simulink model "SvpwmComparisonTest"  (R2026b)
settings: Solver=FixedStepDiscrete  StopTime=svpwmTest.StopTime  FixedStep=svpwmTest.Ts
PostLoadFcn:
  | svpwmDir=fileparts(get_param(bdroot,'FileName'));addpath(fullfile(svpwmDir,'seven_segment'),fullfile(svpwmDir,'five_segment'),fullfile(svpwmDir,'..','..','parameter'));assignin(get_param(bdroot,'ModelWorkspace'),'svpwmTest',svpwm_test_parameters());clear svpwmDir;
model workspace (MAT data in the model file):
  svpwmTest.Ts = 0.0001
  svpwmTest.Stimulus = [0  16.6276877527  9.6  48; 0.0001  1.17566092718e-15  19.2  48; 0.0002  -16.6276877527  9.6  48; 0.0003  -16.6276877527  -9.6  48; 0.0004  -3.52698278154e-15  -19.2  48; 0.0005  16.6276877527  -9.6  48; 0.0006  8.31384387633  4.8  24; 0.0007  5.87830463591e-16  9.6  24; 0.0008  -8.31384387633  4.8  24; 0.0009  -8.31384387633  -4.8  24; 0.001  -1.76349139077e-15  -9.6  24; 0.0011  8.31384387633  -4.8  24; 0.0012  0  0  48; 0.0013  48  0  48]
  svpwmTest.StopTime = 0.0013
libraries: SvpwmFiveSegment x1, SvpwmSevenSegment x1
settings Model: Creator=24322  LastModifiedBy=24322

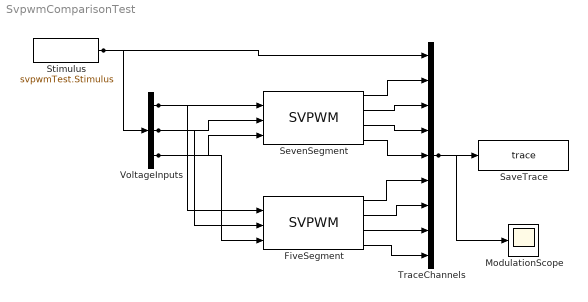
== system SvpwmComparisonTest ==
  FiveSegment : SvpwmFiveSegment/SVPWM  SystemSampleTime=-1  VariantActivationTime=update diagram  EmptyChoice=off  PassThrough=off  PassThroughVariantControl=(default)  EmptyChoiceVariantControl=(default)  AllowFlexibleInterface=on  Latency=0  AutoFrameSizeCalculation=off
  ModulationScope : Scope
  SaveTrace : ToWorkspace  VariableName=trace  SaveFormat=Structure With Time  SampleTime=-1
  SevenSegment : SvpwmSevenSegment/SVPWM  SystemSampleTime=-1  VariantActivationTime=update diagram  EmptyChoice=off  PassThrough=off  PassThroughVariantControl=(default)  EmptyChoiceVariantControl=(default)  AllowFlexibleInterface=on  Latency=0  AutoFrameSizeCalculation=off
  Stimulus : FromWorkspace  VariableName=svpwmTest.Stimulus  SampleTime=svpwmTest.Ts  Interpolate=off  OutputAfterFinalValue=Holding final value
  TraceChannels : Mux  Inputs=9
  VoltageInputs : Demux  Outputs=3
  wires:
  FiveSegment/4 -> TraceChannels/9
  SevenSegment/4 -> TraceChannels/5
  FiveSegment/3 -> TraceChannels/8
  SevenSegment/3 -> TraceChannels/4
  FiveSegment/2 -> TraceChannels/7
  SevenSegment/2 -> TraceChannels/3
  FiveSegment/1 -> TraceChannels/6
  SevenSegment/1 -> TraceChannels/2
  VoltageInputs/3 -> SevenSegment/3, FiveSegment/3
  VoltageInputs/2 -> SevenSegment/2, FiveSegment/2
  VoltageInputs/1 -> SevenSegment/1, FiveSegment/1
  TraceChannels/1 -> ModulationScope/1, SaveTrace/1
  Stimulus/1 -> VoltageInputs/1, TraceChannels/1
